simulink model "Ideal_2ndOrder_StepRes"  (R2013b)
settings: Solver=ode45  StartTime=0.0  StopTime=sim_stop_time  FixedStep=sim_step_size  MaxStep=sim_step_size  RelTol=1e-3
PreLoadFcn:
  | motor_parameters;
  | sim_stop_time = 0.3;
  | sim_step_size = 0.0001;
values from neighbouring files (symbols this model uses):
  b = 0.0006001689451    [Ideal_2ndOrder_PI_Prop_only.mat]    (also in Ideal_2ndOrder_PI_Sat.mat; Ideal_2ndOrder_PI_Sat_CtlStep.mat; Ideal_2ndOrder_PI_Sat_CtlStep_Q.mat; Ideal_2ndOrder_PI_Sat_CtlStep_Q_verification.mat)
  J = 0.001321184025    [Ideal_2ndOrder_PI_Prop_only.mat]    (also in Ideal_2ndOrder_PI_Sat.mat; Ideal_2ndOrder_PI_Sat_CtlStep.mat; Ideal_2ndOrder_PI_Sat_CtlStep_Q.mat; Ideal_2ndOrder_PI_Sat_CtlStep_Q_verification.mat)
  Kb = 0.4952900056    [Ideal_2ndOrder_PI_Prop_only.mat]    (also in Ideal_2ndOrder_PI_Sat.mat; Ideal_2ndOrder_PI_Sat_CtlStep.mat; Ideal_2ndOrder_PI_Sat_CtlStep_Q.mat; Ideal_2ndOrder_PI_Sat_CtlStep_Q_verification.mat)
  Kt = 0.3233728703    [Ideal_2ndOrder_PI_Prop_only.mat]    (also in Ideal_2ndOrder_PI_Sat.mat; Ideal_2ndOrder_PI_Sat_CtlStep.mat; Ideal_2ndOrder_PI_Sat_CtlStep_Q.mat; Ideal_2ndOrder_PI_Sat_CtlStep_Q_verification.mat)
  L = 0.0047    [Ideal_2ndOrder_PI_Prop_only.mat]    (also in Ideal_2ndOrder_PI_Sat.mat; Ideal_2ndOrder_PI_Sat_CtlStep.mat; Ideal_2ndOrder_PI_Sat_CtlStep_Q.mat; Ideal_2ndOrder_PI_Sat_CtlStep_Q_verification.mat)
  R = 5.262773292    [Ideal_2ndOrder_PI_Prop_only.mat]    (also in Ideal_2ndOrder_PI_Sat.mat; Ideal_2ndOrder_PI_Sat_CtlStep.mat; Ideal_2ndOrder_PI_Sat_CtlStep_Q.mat; Ideal_2ndOrder_PI_Sat_CtlStep_Q_verification.mat)
  Vref = 9    [Ideal_2ndOrder_PI_Prop_only.mat]    (also in Ideal_2ndOrder_PI_Sat.mat; Ideal_2ndOrder_PI_Sat_CtlStep.mat; Ideal_2ndOrder_PI_Sat_CtlStep_Q.mat; Ideal_2ndOrder_PI_Sat_CtlStep_Q_verification.mat = 4.5)
settings Model: Creator=nding  LastModifiedBy=nding

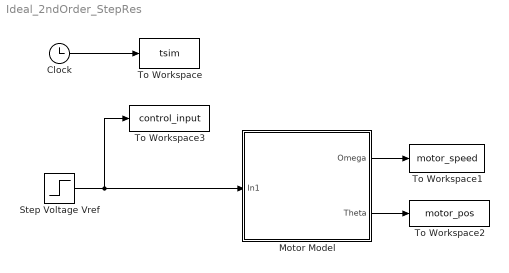
== system Ideal_2ndOrder_StepRes ==
  Clock : Clock
  Motor Model : Subsystem
  Step Voltage Vref : Step  Time=0  After=Vref  SampleTime=0
  To Workspace : ToWorkspace  VariableName=tsim  SampleTime=sim_step_size
  To Workspace1 : ToWorkspace  VariableName=motor_speed  SampleTime=sim_step_size
  To Workspace2 : ToWorkspace  VariableName=motor_pos  SampleTime=sim_step_size
  To Workspace3 : ToWorkspace  VariableName=control_input  SampleTime=sim_step_size
  wires:
  Clock/1 -> To Workspace/1
  Step Voltage Vref/1 -> To Workspace3/1, Motor Model/1(In1)
  Motor Model/1(Omega) -> To Workspace1/1
  Motor Model/2(Theta) -> To Workspace2/1

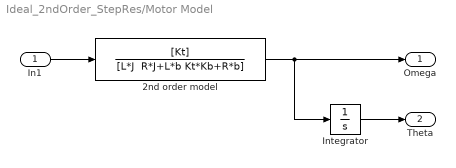
== system Ideal_2ndOrder_StepRes/Motor Model ==
  In1 : Inport
  2nd order model : TransferFcn  Numerator=[Kt]  Denominator="[L*J  R*J+L*b Kt*Kb+R*b]"
  Integrator : Integrator
  Omega : Outport
  Theta : Outport  Port=2
  wires:
  2nd order model/1 -> Omega/1, Integrator/1
  In1/1 -> 2nd order model/1
  Integrator/1 -> Theta/1
